simulink model "student_model_ref"  (R2026a)
settings: Solver=VariableStepAuto  StopTime=t_sim  RelTol=1e-5  EnableMultiTasking=on
values from neighbouring files (symbols this model uses):
  A = [0 1; -wm^2 -2*zm*wm]    [lab3_figures.m]    (also in lab3model.m; modelA.m; modelB.m; modelC.m)
  Ap = [0 1; -wn^2 -2*c.zp*wn]    [lab3_figures.m]    (also in lab3model.m = [0 1; -wn^2 -2*zn*wn]; modelA.m = [0 1; -wn^2 -2*zn*wn]; modelB.m = [0 1; -wn^2 -2*zn*wn]; modelC.m = [0 1; -wn^2 -2*zn*wn])
  B = [0; 1]    [lab3_figures.m]    (also in lab3model.m = [0;1]; modelA.m = [0;1]; modelB.m = [0;1]; modelC.m = [0;1])
  Bp = [0; 1]    [lab3_figures.m]    (also in lab3model.m = [0;1]; modelA.m = [0;1]; modelB.m = [0;1]; modelC.m = [0;1])
  C = eye(2)    [lab3_figures.m]    (also in lab3model.m; modelA.m; modelB.m; modelC.m)
  Cp = eye(2)    [lab3_figures.m]    (also in lab3model.m; modelA.m; modelB.m; modelC.m)
  D = [0; 0]    [lab3_figures.m]    (also in lab3model.m = [0;0]; modelA.m = [0;0]; modelB.m = [0;0]; modelC.m = [0;0])
  Dp = [0; 0]    [lab3_figures.m]    (also in lab3model.m = [0;0]; modelA.m = [0;0]; modelB.m = [0;0]; modelC.m = [0;0])
  t_off = tOff    [lab3_figures.m]    (also in lab3model.m = 5; modelA.m = 5; modelB.m = 5; modelC.m = 5)
  t_on = tOn    [lab3_figures.m]    (also in lab3model.m = 1; modelA.m = 1; modelB.m = 1; modelC.m = 1)
undefined symbols (not defined in the file or in its folder): student_model_ref_controller
settings Model: Creator=Kelvin  LastModifiedBy=noahtouchton
settings DataIOCC: SignalLoggingSaveFormat=ModelDataLogs
settings DebuggingCC: UnderspecifiedInitializationDetection=Classic
settings HardwareCC: ProdHWDeviceType=32-bit Generic
settings GRTTargetCC: CombineOutputUpdateFcns=off  GRTInterface=on

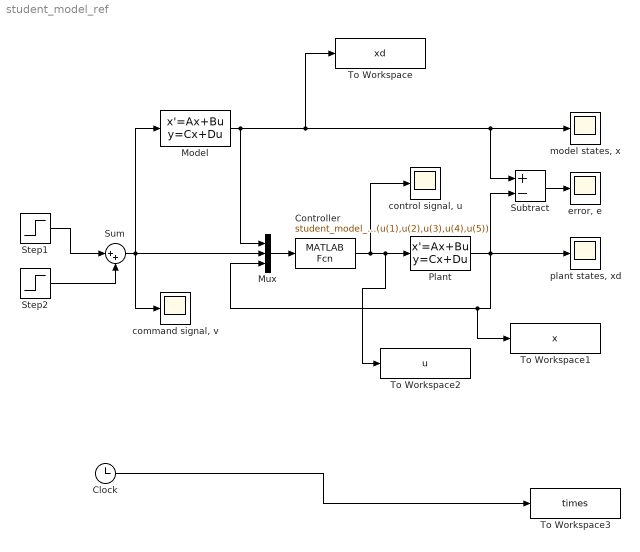
== system student_model_ref ==
  Clock : Clock
  Controller : MATLABFcn  MATLABFcn=student_model_ref_controller(u(1),u(2),u(3),u(4),u(5))
  Model : StateSpace  A=A  B=B  C=C  D=D  InitialCondition=0
  Mux : Mux  Inputs=3
  Plant : StateSpace  A=Ap  B=Bp  C=Cp  D=Dp  InitialCondition=0
  Step1 : Step  Time=t_on  FinalValue=step1  SampleTime=0  ZeroCross=off
  Step2 : Step  Time=t_off  FinalValue=step2  SampleTime=0  ZeroCross=off
  Subtract : Sum  Inputs=+-
  Sum : Sum  Inputs=|++
  To Workspace : ToWorkspace  VariableName=xd  SaveFormat=Timeseries  SampleTime=-1
  To Workspace1 : ToWorkspace  VariableName=x  SampleTime=-1
  To Workspace2 : ToWorkspace  VariableName=u  SaveFormat=Timeseries  SampleTime=-1
  To Workspace3 : ToWorkspace  VariableName=times  SaveFormat=Timeseries  SampleTime=-1
  "command signal, v" : Scope
      settings: DataLoggingVariableName=ScopeData4
  "control signal, u" : Scope
      settings: TimeSpan=10  ActiveDisplayYMinimum=0  ActiveDisplayYMaximum=0.35  DataLoggingVariableName=ScopeData3
  "error, e" : Scope
      settings: DataLoggingVariableName=ScopeData2
  "model states, x" : Scope
      settings: TimeSpan=10  ActiveDisplayYMinimum=0  ActiveDisplayYMaximum=0.02
  "plant states, xd" : Scope
      settings: TimeSpan=10  ActiveDisplayYMinimum=-0.005  ActiveDisplayYMaximum=0.02
  wires:
  Sum/1 -> Mux/2, "command signal, v"/1, Model/1
  Mux/1 -> Controller/1
  Controller/1 -> "control signal, u"/1, To Workspace2/1, Plant/1
  Plant/1 -> To Workspace1/1, Mux/3, "plant states, xd"/1, Subtract/2
  Model/1 -> Mux/1, To Workspace/1, Subtract/1, "model states, x"/1
  Subtract/1 -> "error, e"/1
  Step1/1 -> Sum/1
  Step2/1 -> Sum/2
  Clock/1 -> To Workspace3/1
